simulink library "Lib_Piccolo"  (R2018b)
settings: Solver=VariableStepAuto  StartTime=0.0  StopTime=10.0  RelTol=1e-3
values from neighbouring files (symbols this model uses):
  AccelErrInt2Brakes = 0.15    [SimulationControlConfig16P.m]    (also in SimulationControlConfig16P_LEGACY.m; SimulationControlConfigTAILLESS.m = 0.2; SimulationControlConfigUTAIL.m = 0.2)
  AileronMax = 25    [SimulationControlConfig16P.m]    (also in SimulationControlConfig16P_LEGACY.m; SimulationControlConfigTAILLESS.m; SimulationControlConfigUTAIL.m)
  AileronPower = 0.00268    [SimulationControlConfig16P.m]    (also in SimulationControlConfig16P_LEGACY.m; SimulationControlConfigTAILLESS.m; SimulationControlConfigUTAIL.m)
  AileronSurfaceMax = 45    [SimulationControlConfig16P.m]    (also in SimulationControlConfig16P_LEGACY.m)
  AileronTrim = 0    [SimulationControlConfig16P.m]    (also in SimulationControlConfig16P_LEGACY.m; SimulationControlConfigTAILLESS.m; SimulationControlConfigUTAIL.m)
  Alt = 1000 + TerrainHeight    [SimulationStateConfig.m]
  AltCruise_m = testPlans(testIndx).terrainElevation * 0.3048 + 200    [SimulationControlConfig16P.m]    (also in SimulationControlConfigTAILLESS.m = 1083; SimulationControlConfigUTAIL.m = testPlans(testIndx).terrainElevation * 0.3048 + 152)
  AltitudeRate2PitchCmdIntegratorInit = 0.1    [SimulationControlPre.m]
  AltMax = 10000    [SimulationControlConfig16P.m]    (also in SimulationControlConfig16P_LEGACY.m; SimulationControlConfigTAILLESS.m; SimulationControlConfigUTAIL.m)
  AltMaxAccel = 1.25    [SimulationControlConfig16P.m]    (also in SimulationControlConfig16P_LEGACY.m = 0.9; SimulationControlConfigTAILLESS.m = 1.7; SimulationControlConfigUTAIL.m = 2)
  AltMin = 0    [SimulationControlConfig16P.m]    (also in SimulationControlConfig16P_LEGACY.m; SimulationControlConfigTAILLESS.m; SimulationControlConfigUTAIL.m)
  AltRateCmd2Pitch = 0.50    (= 0.5)    [SimulationControlConfig16P.m]    (also in SimulationControlConfig16P_LEGACY.m = 0.6; SimulationControlConfigTAILLESS.m = 0.2; SimulationControlConfigUTAIL.m = 0.3)
  AltRateError2Pitch = 0.40    (= 0.4)    [SimulationControlConfig16P.m]    (also in SimulationControlConfig16P_LEGACY.m; SimulationControlConfigTAILLESS.m = 0.55; SimulationControlConfigUTAIL.m = 0.55)
  AltRateErrorInt2Pitch = 0.50    (= 0.5)    [SimulationControlConfig16P.m]    (also in SimulationControlConfig16P_LEGACY.m = 0.45; SimulationControlConfigTAILLESS.m; SimulationControlConfigUTAIL.m = 0.75)
  AltRateLpfCutOff = 3    [SimulationControlConfig16P.m]    (also in SimulationControlConfig16P_LEGACY.m; SimulationControlConfigTAILLESS.m = 2; SimulationControlConfigUTAIL.m = 2)
  AutoNosegear2Rudder = 26    [SimulationControlConfig16P.m]    (also in SimulationControlConfig16P_LEGACY.m; SimulationControlConfigTAILLESS.m = 25.2; SimulationControlConfigUTAIL.m = 14)
  b = 5.54    [SimulationControlConfig16P.m]    (also in SimulationControlConfig16P_LEGACY.m; SimulationControlConfigTAILLESS.m = 2.37; SimulationControlConfigUTAIL.m = 2.37)
  Bank2AileronIntegratorInit = 0    [SimulationControlPre.m]
  BankMax_User = BankMax_User/180*pi    (= 0.523598775598)    [SimulationControlConfig16P.m]    (also in SimulationControlConfig16P_LEGACY.m; SimulationControlConfigTAILLESS.m = 0.610865238198; SimulationControlConfigUTAIL.m = 0.628318530718)
  baseLegFlaps = 20    [SimulationControlConfig16P.m]    (also in SimulationControlConfig16P_LEGACY.m = 0; SimulationControlConfigTAILLESS.m = 15; SimulationControlConfigUTAIL.m = 10)
  C = GeneticOpt.C    [SimulationCostFunction.m]
  c = Sw/b    (= 0.841696750903)    [SimulationControlConfig16P.m]    (also in SimulationControlConfig16P_LEGACY.m; SimulationControlConfigTAILLESS.m = 0.354008438819; SimulationControlConfigUTAIL.m = 0.354008438819)
  cell2WheelFactorMG = 5.98    [SimulationSensorConfig16P_LEGACY.m]
  cell2WheelFactorNG = 1    [SimulationSensorConfig16P_LEGACY.m]
  cellSatMaxMG = 15000    [SimulationSensorConfig16P.m]    (also in SimulationSensorConfig16P_LEGACY.m; SimulationSensorConfigTAILLESS7P.m; SimulationSensorConfigUTAIL7P.m)
  cellSatMaxNG = 1000    [SimulationSensorConfig16P.m]    (also in SimulationSensorConfig16P_LEGACY.m; SimulationSensorConfigTAILLESS7P.m; SimulationSensorConfigUTAIL7P.m)
  cellSatMinMG = -15000    [SimulationSensorConfig16P.m]    (also in SimulationSensorConfig16P_LEGACY.m; SimulationSensorConfigTAILLESS7P.m; SimulationSensorConfigUTAIL7P.m)
  cellSatMinNG = -1000    [SimulationSensorConfig16P.m]    (also in SimulationSensorConfig16P_LEGACY.m; SimulationSensorConfigTAILLESS7P.m; SimulationSensorConfigUTAIL7P.m)
  CL_Limit = CL_Max    (= 0.54)    [SimulationControlConfig16P.m]    (also in SimulationControlConfig16P_LEGACY.m; SimulationControlConfigTAILLESS.m; SimulationControlConfigUTAIL.m = 0.53)
  CL_Max = 0.54    [SimulationControlConfig16P.m]    (also in SimulationControlConfig16P_LEGACY.m; SimulationControlConfigTAILLESS.m; SimulationControlConfigUTAIL.m = 0.53)
  CL_Max_Nom = 0.465    [SimulationControlConfig16P.m]    (also in SimulationControlConfig16P_LEGACY.m; SimulationControlConfigTAILLESS.m = 0.39; SimulationControlConfigUTAIL.m)
  CL_Min = 0    [SimulationControlConfig16P.m]    (also in SimulationControlConfig16P_LEGACY.m; SimulationControlConfigTAILLESS.m; SimulationControlConfigUTAIL.m)
  ClimbMaxFraction = 0.35    [SimulationControlConfig16P.m]    (also in SimulationControlConfig16P_LEGACY.m = 0.24; SimulationControlConfigTAILLESS.m = 0.19; SimulationControlConfigUTAIL.m = 0.21)
  ClimboutMaxBank = 7.0    (= 7)    [SimulationControlConfig16P.m]    (also in SimulationControlConfig16P_LEGACY.m; SimulationControlConfigTAILLESS.m = 5; SimulationControlConfigUTAIL.m)
  ClimboutTimer = 7.0    (= 7)    [SimulationControlConfig16P.m]    (also in SimulationControlConfig16P_LEGACY.m; SimulationControlConfigTAILLESS.m; SimulationControlConfigUTAIL.m)
  dCl_per_dFlap = 0.005581818    [SimulationControlConfig16P.m]    (also in SimulationControlConfig16P_LEGACY.m = 0; SimulationControlConfigTAILLESS.m = 0; SimulationControlConfigUTAIL.m = 0)
  DecelerationCmd = 3.1    [SimulationControlConfig16P.m]    (also in SimulationControlConfig16P_LEGACY.m; SimulationControlConfigTAILLESS.m = 0.1; SimulationControlConfigUTAIL.m = 0.1)
  DeRotateLogicEndTimer = abs((NoseDownLimit_Deg-1)/DeRotateRamp_Dps)    [SimulationControlConfig16P.m]    (also in SimulationControlConfig16P_LEGACY.m; SimulationControlConfigTAILLESS.m; SimulationControlConfigUTAIL.m)
  DeRotateLogicHoldNoseUpTimer = 0.1    [SimulationControlConfig16P.m]    (also in SimulationControlConfig16P_LEGACY.m; SimulationControlConfigTAILLESS.m; SimulationControlConfigUTAIL.m)
  DeRotateLogicTimerTimeout = 2    [SimulationControlConfig16P.m]    (also in SimulationControlConfig16P_LEGACY.m; SimulationControlConfigTAILLESS.m; SimulationControlConfigUTAIL.m)
  DeRotateLowerCmdSaturation = 0    [SimulationControlConfig16P.m]    (also in SimulationControlConfig16P_LEGACY.m; SimulationControlConfigTAILLESS.m; SimulationControlConfigUTAIL.m)
  DeRotateRamp_Dps = 3    [SimulationControlConfig16P.m]    (also in SimulationControlConfig16P_LEGACY.m; SimulationControlConfigTAILLESS.m = 8; SimulationControlConfigUTAIL.m = 8)
  DeRotateUpperCmdSaturation = 7    [SimulationControlConfig16P.m]    (also in SimulationControlConfig16P_LEGACY.m; SimulationControlConfigTAILLESS.m; SimulationControlConfigUTAIL.m)
  DescentMaxFraction = 0.22    [SimulationControlConfig16P.m]    (also in SimulationControlConfig16P_LEGACY.m = 0.2; SimulationControlConfigTAILLESS.m = 0.17; SimulationControlConfigUTAIL.m = 0.17)
  DesktopSimTerrainOffset_m = 0.406    [SimulationAircraftConfig.m]
  downwindFlaps = 0    [SimulationControlConfig16P.m]    (also in SimulationControlConfig16P_LEGACY.m; SimulationControlConfigTAILLESS.m; SimulationControlConfigUTAIL.m)
  DP_init = 0.5*1.225*V_init^2    [SimulationControlConfig16P.m]    (also in SimulationControlConfig16P_LEGACY.m; SimulationControlConfigTAILLESS.m; SimulationControlConfigUTAIL.m)
  dscNoiseMG = 1    [SimulationSensorConfig16P_LEGACY.m]
  dscNoiseNG = 0.25    [SimulationSensorConfig16P_LEGACY.m]
  DSCnumBits = 24    [SimulationSensorConfig16P.m]    (also in SimulationSensorConfig16P_LEGACY.m; SimulationSensorConfigTAILLESS7P.m; SimulationSensorConfigUTAIL7P.m)
  DSCRangeMaxMG = 15000    [SimulationSensorConfig16P.m]    (also in SimulationSensorConfig16P_LEGACY.m; SimulationSensorConfigTAILLESS7P.m; SimulationSensorConfigUTAIL7P.m)
  DSCRangeMaxNG = 1000    [SimulationSensorConfig16P.m]    (also in SimulationSensorConfig16P_LEGACY.m; SimulationSensorConfigTAILLESS7P.m; SimulationSensorConfigUTAIL7P.m)
  DSCRangeMinMG = -15000    [SimulationSensorConfig16P.m]    (also in SimulationSensorConfig16P_LEGACY.m; SimulationSensorConfigTAILLESS7P.m; SimulationSensorConfigUTAIL7P.m)
  DSCRangeMinNG = -1000    [SimulationSensorConfig16P.m]    (also in SimulationSensorConfig16P_LEGACY.m; SimulationSensorConfigTAILLESS7P.m; SimulationSensorConfigUTAIL7P.m)
  dt = DLLSim.dt    [SimulationTimeStep.m]    (also in SimulationTrim.m = 0.02)
  EarlyTouchdownThreshold = 3.0    (= 3)    [SimulationControlConfig16P.m]    (also in SimulationControlConfig16P_LEGACY.m; SimulationControlConfigTAILLESS.m = 2.2; SimulationControlConfigUTAIL.m = 2.5)
  ElevatorDeflectionRate = 15    [SimulationControlConfig16P.m]    (also in SimulationControlConfig16P_LEGACY.m = 12; SimulationControlConfigTAILLESS.m = 10; SimulationControlConfigUTAIL.m = 12)
  ElevatorMax = 25    [SimulationControlConfig16P.m]    (also in SimulationControlConfig16P_LEGACY.m; SimulationControlConfigTAILLESS.m; SimulationControlConfigUTAIL.m)
  ElevatorPower = -0.002209    [SimulationControlConfig16P.m]    (also in SimulationControlConfig16P_LEGACY.m; SimulationControlConfigTAILLESS.m = -0.002956; SimulationControlConfigUTAIL.m = -0.00205983)
  ElevatorTrim = -3.5    [SimulationControlConfig16P.m]    (also in SimulationControlConfig16P_LEGACY.m; SimulationControlConfigTAILLESS.m = -6; SimulationControlConfigUTAIL.m = -8)
  elevonBias = 0    [SimulationControlConfig16P.m]    (also in SimulationControlConfig16P_LEGACY.m; SimulationControlConfigTAILLESS.m; SimulationControlConfigUTAIL.m)
  Enable_TAS_Protection = 0    [SimulationControlConfig16P.m]    (also in SimulationControlConfig16P_LEGACY.m; SimulationControlConfigTAILLESS.m; SimulationControlConfigUTAIL.m)
  EnableCrossTrackAbort = 1    [SimulationControlConfig16P.m]    (also in SimulationControlConfigTAILLESS.m; SimulationControlConfigUTAIL.m)
  EnergyBandwidth = 0.02    [SimulationControlConfig16P.m]    (also in SimulationControlConfig16P_LEGACY.m; SimulationControlConfigTAILLESS.m = 0.06; SimulationControlConfigUTAIL.m = 0.06)
  EngineLhFuelCut = 0    [SimulationAircraftConfig.m]
  EngineRhFuelCut = 0    [SimulationAircraftConfig.m]
  FastThrottleRate = 0.075    [SimulationControlConfig16P.m]    (also in SimulationControlConfig16P_LEGACY.m = 0.05; SimulationControlConfigTAILLESS.m = 0.1; SimulationControlConfigUTAIL.m = 0.1)
  FilterWarmUpTime = 2    [SimulationSensorConfig16P.m]    (also in SimulationSensorConfig16P_LEGACY.m; SimulationSensorConfigTAILLESS7P.m; SimulationSensorConfigUTAIL7P.m)
  finalApproachFlaps = 20    [SimulationControlConfig16P.m]    (also in SimulationControlConfig16P_LEGACY.m = 0; SimulationControlConfigTAILLESS.m = 22; SimulationControlConfigUTAIL.m = 10)
  FinalDescentSlope_Deg = testPlans(testIndx).descentSlope    [SimulationControlConfig16P.m]    (also in SimulationControlConfig16P_LEGACY.m; SimulationControlConfigTAILLESS.m; SimulationControlConfigUTAIL.m)
  flapMax = 0    [SimulationControlConfig16P.m]    (also in SimulationControlConfig16P_LEGACY.m; SimulationControlConfigTAILLESS.m; SimulationControlConfigUTAIL.m)
  flapRate = 7.5    [SimulationControlConfig16P.m]    (also in SimulationControlConfig16P_LEGACY.m; SimulationControlConfigTAILLESS.m = 6.6; SimulationControlConfigUTAIL.m)
  FlareHeight = 5    [SimulationControlConfig16P.m]    (also in SimulationControlConfig16P_LEGACY.m = 4.8; SimulationControlConfigTAILLESS.m = 2.5; SimulationControlConfigUTAIL.m = 2)
  FlareVerticalRate_mps = -0.4    [SimulationControlConfig16P.m]    (also in SimulationControlConfig16P_LEGACY.m = -0.5; SimulationControlConfigTAILLESS.m = -0.15; SimulationControlConfigUTAIL.m = -0.15)
  Fp_Aileron = 0.55*2*pi*RollRateLpfCutoff*dt    [SimulationControlConfig16P.m]    (also in SimulationControlConfig16P_LEGACY.m; SimulationControlConfigTAILLESS.m; SimulationControlConfigUTAIL.m)
  Fp_Alt = 0.55*AltBandwidth    (= 0.099)    [SimulationControlConfig16P.m]    (also in SimulationControlConfig16P_LEGACY.m; SimulationControlConfigTAILLESS.m = 0.587477826221; SimulationControlConfigUTAIL.m = 0.69115038379)
  Fp_AltRate = 0.55*2*pi*AltRateLpfCutOff*dt    [SimulationControlConfig16P.m]    (also in SimulationControlConfig16P_LEGACY.m; SimulationControlConfigTAILLESS.m; SimulationControlConfigUTAIL.m)
  Fp_Elevator = 0.55*2*pi*PitchRateLpfCutoff*dt    [SimulationControlConfig16P.m]    (also in SimulationControlConfig16P_LEGACY.m; SimulationControlConfigTAILLESS.m; SimulationControlConfigUTAIL.m)
  Fp_Energy = 0.55*2*pi*EnergyBandwidth    (= 0.069115038379)    [SimulationControlConfig16P.m]    (also in SimulationControlConfig16P_LEGACY.m; SimulationControlConfigTAILLESS.m = 0.207345115137; SimulationControlConfigUTAIL.m = 0.207345115137)
  Fp_Energy2 = 0.55*2*pi*EnergyBandwidth*dt    [SimulationControlConfig16P.m]    (also in SimulationControlConfig16P_LEGACY.m; SimulationControlConfigTAILLESS.m; SimulationControlConfigUTAIL.m)
  Fp_Pitch = 0.55*2*pi*PitchBandwidth    (= 2.76460153516)    [SimulationControlConfig16P.m]    (also in SimulationControlConfig16P_LEGACY.m = 3.11017672705; SimulationControlConfigTAILLESS.m = 3.80132711084; SimulationControlConfigUTAIL.m = 2.41902634326)
  Fp_Pitch_2 = 0.55*2*pi*PitchBandwidth*dt    [SimulationControlConfig16P.m]    (also in SimulationControlConfig16P_LEGACY.m; SimulationControlConfigTAILLESS.m; SimulationControlConfigUTAIL.m)
  Fp_Roll = RollBandwidth^2    (= 1)    [SimulationControlConfig16P.m]    (also in SimulationControlConfig16P_LEGACY.m = 1.44; SimulationControlConfigTAILLESS.m; SimulationControlConfigUTAIL.m)
  Fp_Rudder = 0.55*2*pi*YawRateLpfCutoff*dt    [SimulationControlConfig16P.m]    (also in SimulationControlConfig16P_LEGACY.m; SimulationControlConfigTAILLESS.m; SimulationControlConfigUTAIL.m)
  Fp_TAS = 0.55*2*pi*TASBandwidth    (= 0.103672557568)    [SimulationControlConfig16P.m]    (also in SimulationControlConfig16P_LEGACY.m; SimulationControlConfigTAILLESS.m = 0.172787595947; SimulationControlConfigUTAIL.m = 0.172787595947)
  Fp_TAS_Filter = 2*pi*TasLpfCutoff*dt    [SimulationControlConfig16P.m]    (also in SimulationControlConfig16P_LEGACY.m; SimulationControlConfigTAILLESS.m; SimulationControlConfigUTAIL.m)
  Fp_Turn = 0.55*2*pi*TurnErrLPFcutoff    (= 0.0345575191895)    [SimulationControlConfig16P.m]    (also in SimulationControlConfig16P_LEGACY.m; SimulationControlConfigTAILLESS.m = 0.172787595947; SimulationControlConfigUTAIL.m = 0.172787595947)
  Fp_TurnDerr = 0.55*2*pi*TurnDerivativeLPFcutoff    (= 0.0345575191895)    [SimulationControlConfig16P.m]    (also in SimulationControlConfig16P_LEGACY.m; SimulationControlConfigTAILLESS.m = 0.172787595947; SimulationControlConfigUTAIL.m = 0.172787595947)
  FTV = 3    [SimulationAircraftConfig.m]
  ftvStaticPositionError = 1/1.18    (= 0.847457627119)    [SimulationSensorConfig16P.m]    (also in SimulationSensorConfig16P_LEGACY.m; SimulationSensorConfigTAILLESS7P.m = 1; SimulationSensorConfigUTAIL7P.m = 1)
  g = 9.81    [SimulationStateConfig.m]
  GustSpd_Kts = testPlans(testIndx).gustSpd    [SimulationStateConfig.m]
  GustTriggerVal = testPlans(testIndx).gustTriggerVal    [SimulationStateConfig.m]
  HeadingErr2TurnRate = 0.5    [SimulationControlConfig16P.m]    (also in SimulationControlConfig16P_LEGACY.m; SimulationControlConfigTAILLESS.m; SimulationControlConfigUTAIL.m)
  HeadingErrDer2TurnRate = 0.3    [SimulationControlConfig16P.m]    (also in SimulationControlConfig16P_LEGACY.m; SimulationControlConfigTAILLESS.m; SimulationControlConfigUTAIL.m)
  IASbounce = IASstall*0.8    [SimulationControlPre.m]
  IAScruiseCMD = sqrt(2*m*9.81/(1.225*Sw*CL_cruise))    [SimulationControlConfig16P.m]    (also in SimulationControlConfig16P_LEGACY.m; SimulationControlConfigTAILLESS.m; SimulationControlConfigUTAIL.m)
  IASfinalCMD = 1.12 * IASmin    [SimulationControlConfig16P.m]    (also in SimulationControlConfig16P_LEGACY.m = 1.10 * IASmin; SimulationControlConfigTAILLESS.m = 1.10 * IASmin; SimulationControlConfigUTAIL.m = 1.15 * IASmin)
  IASflareCMD = IASstall    [SimulationControlConfig16P.m]    (also in SimulationControlConfig16P_LEGACY.m; SimulationControlConfigTAILLESS.m; SimulationControlConfigUTAIL.m)
  IASmax = 64    [SimulationControlConfig16P.m]    (also in SimulationControlConfig16P_LEGACY.m = 46; SimulationControlConfigTAILLESS.m = 38.58; SimulationControlConfigUTAIL.m = 35)
  IASmin = sqrt(2*m*9.81/(1.225*Sw*0.9*CL_Max_Nom))    [SimulationControlConfig16P.m]    (also in SimulationControlConfig16P_LEGACY.m; SimulationControlConfigTAILLESS.m; SimulationControlConfigUTAIL.m)
  IASshortCMD = IASstall    [SimulationControlConfig16P.m]    (also in SimulationControlConfig16P_LEGACY.m; SimulationControlConfigTAILLESS.m; SimulationControlConfigUTAIL.m)
  IASstall = sqrt(2*m*9.81/(1.225*Sw*CL_Max))    [SimulationControlConfig16P.m]    (also in SimulationControlConfig16P_LEGACY.m; SimulationControlConfigTAILLESS.m; SimulationControlConfigUTAIL.m)
  inFlight = 1    [SimulationControlConfig16P.m]    (also in SimulationControlConfigTAILLESS.m; SimulationControlConfigUTAIL.m)
  JetCatOffset = 5    [SimulationControlConfig16P.m]    (also in SimulationControlConfig16P_LEGACY.m)
  LaunchRollingElevator = -1.5    [SimulationControlConfig16P.m]    (also in SimulationControlConfig16P_LEGACY.m; SimulationControlConfigTAILLESS.m = 1; SimulationControlConfigUTAIL.m = 1)
  ldg_NosegearMax = 10    [SimulationControlConfig16P.m]    (also in SimulationControlConfig16P_LEGACY.m; SimulationControlConfigTAILLESS.m; SimulationControlConfigUTAIL.m)
  ldg_TrackVyErrInt2Nosegear = 0.1250    (= 0.125)    [SimulationControlConfig16P.m]    (also in SimulationControlConfig16P_LEGACY.m; SimulationControlConfigTAILLESS.m = 0.00714285714286; SimulationControlConfigUTAIL.m = 0.00714285714286)
  ldg_TrackVyErrPro2Nosegear = 0.35    [SimulationControlConfig16P.m]    (also in SimulationControlConfig16P_LEGACY.m; SimulationControlConfigTAILLESS.m = 0.0546666666667; SimulationControlConfigUTAIL.m = 0.0546666666667)
  ldg_TrackY2Vy = 0.07    [SimulationControlConfig16P.m]    (also in SimulationControlConfig16P_LEGACY.m; SimulationControlConfigTAILLESS.m = 0.17; SimulationControlConfigUTAIL.m = 0.17)
  ldg_Vy2NosegearScalingPower = 1.075    [SimulationControlConfig16P.m]    (also in SimulationControlConfig16P_LEGACY.m; SimulationControlConfigTAILLESS.m = 0.6; SimulationControlConfigUTAIL.m = 0.5)
  ldg_Y2VyScalingPower = 0.175    [SimulationControlConfig16P.m]    (also in SimulationControlConfig16P_LEGACY.m; SimulationControlConfigTAILLESS.m = 0; SimulationControlConfigUTAIL.m = 0)
  ldg_YawRate2Nosegear = 0.175    [SimulationControlConfig16P.m]    (also in SimulationControlConfig16P_LEGACY.m; SimulationControlConfigTAILLESS.m = 0.065; SimulationControlConfigUTAIL.m = 0.065)
  LiftSlope = 0.064285    [SimulationControlConfig16P.m]    (also in SimulationControlConfig16P_LEGACY.m; SimulationControlConfigTAILLESS.m = 0.058631; SimulationControlConfigUTAIL.m)
  LPFaileronInit = 0    [SimulationControlPre.m]
  LPFclestInit = 0    [SimulationControlPre.m]
  LPFenergyFFInit = 0    [SimulationControlPre.m]
  LPFtasInit = V_init + 2    [SimulationControlPre.m]
  LPFthrottleInit = ThrottleTrim    [SimulationControlPre.m]
  LPFturnErrInit = 0    [SimulationControlPre.m]
  ... (+115 more)
undefined symbols (not defined in the file or in its folder): abortFlag, alphaHPF, apmDelay, BRWNOUT, CRAWOR, CRAWUR, DiscIntNeverNeededParam, DLLSim, DLLSimStep, ECOMOR, ECOMUR, Fp_Tas, GustTrigger_HeightAgl_m, IPSTAT, LCINTEG, Ldg_Persist_Time, LOWER_FLAGS, MSG_ENABLE, NoiseStd, OLDVAL, OVERRIDE_ENABLE, OVERRIDE_VALUE, REBOOT, reversionEnable, revIASMax, revIASMin, revPitchMax, revPitchMin, revPitchRateMax, revRollMax, revRollRateMax, SAMPLE, SCALON, SensorModel, sigbuilder_block, Sim_Vx, Sim_Vy, Sim_Vz, Sim_Xpos, Sim_Ypos, Sim_Zpos, SYSOR, SYSUR, TARE, TEMPOR, TEMPUR, testIndx, testPlan, testPlans, Trim_piccoloInCmd, Trim_REFSI_FD_IN_nmodeCgShifterCmd_Ft, Trim_REFSI_FD_IN_nmodeFlapLhIBCmd_Deg, Trim_REFSI_FD_IN_nmodeFlapLhOBCmd_Deg, Trim_REFSI_FD_IN_nmodeFlapRhIBCmd_Deg, Trim_REFSI_FD_IN_nmodeFlapRhOBCmd_Deg, Trim_REFSI_FD_IN_nmodeSlatLhCmd_Deg, Trim_REFSI_FD_IN_nmodeSlatRhCmd_Deg, Trim_REFSI_FD_IN_nmodeSplrLhInbdCmd_Deg, Trim_REFSI_FD_IN_nmodeSplrLhOutbdCmd_Deg ... (+5)
libraries: simulink x866, aerolibconvert2 x60, $bdroot x52, aerolibatmos2 x5, dspswit3 x5, simulink_extras x4, dsparch4 x2, Lib_Piccolo_Alt x2, eeGeneralControl x1, dspindex x1
(part 40 of 44)

== system Lib_Piccolo/Ground Detection Systems/WoW Wrapper/Variant Subsystem/Load Cell WoW Model 20/WOW Module/Bias Filters ==
  WOW_NG_RAW_N : Inport
  WOW_MGL_RAW_N : Inport  Port=2
  WOW_MGR_RAW_N : Inport  Port=3
  Bus Creator : BusCreator  Inputs=3
  Ground : Ground
  LPF MGL : Subsystem  mask{Cutoff=SensorModel.WOW.Cell.fc, Init=0}
      mask prompts: Cutoff "Cutoff Frequency [Hz]"; Init "Initial Condition"
  LPF MGR : Subsystem  mask{Cutoff=SensorModel.WOW.Cell.fc, Init=0}
      mask prompts: Cutoff "Cutoff Frequency [Hz]"; Init "Initial Condition"
  LPF NG : Subsystem  mask{Cutoff=SensorModel.WOW.Cell.fc, Init=0}
      mask prompts: Cutoff "Cutoff Frequency [Hz]"; Init "Initial Condition"
  WOW_Bias_Filt_N : Outport  VectorParamsAs1DForOutWhenUnconnected=on
  wires:
  WOW_NG_RAW_N/1 -> LPF NG/1("Input ")
  Bus Creator/1 -> WOW_Bias_Filt_N/1
  LPF NG/1("Output ") -> Bus Creator/1  "Bias_NG_N"
  Ground/1 -> LPF MGL/2(Reset), LPF MGR/2(Reset), LPF NG/2(Reset)
  WOW_MGL_RAW_N/1 -> LPF MGL/1("Input ")
  LPF MGL/1("Output ") -> Bus Creator/2  "Bias_MGL_N"
  LPF MGR/1("Output ") -> Bus Creator/3  "Bias_MGR_N"
  WOW_MGR_RAW_N/1 -> LPF MGR/1("Input ")

== system Lib_Piccolo/Ground Detection Systems/WoW Wrapper/Variant Subsystem/Load Cell WoW Model 20/WOW Module/Command Processing ==
  User Cmd Bus In : Inport
  Bus Selector : BusSelector  OutputSignals=MSG_ENABLE,TARE,OVERRIDE_ENABLE,OVERRIDE_VALUE
  Edge Detector : dspswit3/Edge Detector  InputProcessing=Columns as channels (frame based)
      settings: SourceProductName=DSP System Toolbox  SourceProductBaseCode=DS
  TARE_TRIGGER : Outport
  MSG_ENABLE : Outport  Port=2
  OVERRIDE_ENABLE : Outport  Port=3  OutDataTypeStr=boolean  VectorParamsAs1DForOutWhenUnconnected=on
  OVERRIDE_VALUE : Outport  Port=4  OutDataTypeStr=boolean  VectorParamsAs1DForOutWhenUnconnected=on
  User Cmd Bus Out : Outport  Port=5
  wires:
  Bus Selector/1 -> MSG_ENABLE/1  "<MSG_ENABLE>"
  User Cmd Bus In/1 -> Bus Selector/1, User Cmd Bus Out/1
  Bus Selector/2 -> Edge Detector/1  "<TARE>"
  Edge Detector/1 -> TARE_TRIGGER/1
  Bus Selector/3 -> OVERRIDE_ENABLE/1  "<OVERRIDE_ENABLE>"
  Bus Selector/4 -> OVERRIDE_VALUE/1  "<OVERRIDE_VALUE>"

== system Lib_Piccolo/Ground Detection Systems/WoW Wrapper/Variant Subsystem/Load Cell WoW Model 20/WOW Module/Flag Latch ==
  note: Latch failure/disable state if AP mode is <= climbout, or >= final
  INIT : Inport
  OUTPUT_DISABLE : Inport  Port=2
  PIC_AP_MODE : Inport  Port=3
  Latch : Subsystem
  Latch Activation on Mode : Subsystem
  OR5 : Logic  Operator=OR  IconShape=distinctive  AllPortsSameDT=off  OutDataTypeStr=boolean
  OUTPUT_DISABLE_LATCHED : Outport
  wires:
  INIT/1 -> OR5/1
  Latch/1(Q_Latched) -> OUTPUT_DISABLE_LATCHED/1
  OUTPUT_DISABLE/1 -> OR5/2
  OR5/1 -> Latch/1(D)
  PIC_AP_MODE/1 -> Latch Activation on Mode/1(Piccolo Mode)
  Latch Activation on Mode/1(Mode Latch) -> Latch/2(Enable/!Rst)

== system Lib_Piccolo/Ground Detection Systems/WoW Wrapper/Variant Subsystem/Load Cell WoW Model 20/WOW Module/LPF MGL ==
  "Input " : Inport
  Reset : Inport  Port=2
  Add1 : Sum  Inputs=++|
  Compare To Constant2 : simulink/Logic and Bit Operations/Compare To Constant  relop=>  const=0  OutDataTypeStr=uint8
  Constant11 : Constant  Value=Cutoff
  Resettable Delay : Delay  DelayLength=1  InitialConditionSource=Input port  ExternalReset=Level hold
      settings: InputPortMap=u0,r5,p4
  Switch1 : Switch  Criteria=u2 > Threshold
  a1 : Gain  Gain=SensorModel.WOW.Cell.a1
  b0 : Gain  Gain=SensorModel.WOW.Cell.b0
  "Output " : Outport
  wires:
  Resettable Delay/1 -> a1/1
  b0/1 -> Add1/2
  Add1/1 -> Resettable Delay/1, Switch1/1
  a1/1 -> Add1/1
  "Input "/1 -> b0/1, Switch1/3, Resettable Delay/3
  Switch1/1 -> "Output "/1
  Compare To Constant2/1 -> Switch1/2
  Constant11/1 -> Compare To Constant2/1
  Reset/1 -> Resettable Delay/2

== system Lib_Piccolo/Ground Detection Systems/WoW Wrapper/Variant Subsystem/Load Cell WoW Model 20/WOW Module/LPF MGR ==
  "Input " : Inport
  Reset : Inport  Port=2
  Add1 : Sum  Inputs=++|
  Compare To Constant2 : simulink/Logic and Bit Operations/Compare To Constant  relop=>  const=0  OutDataTypeStr=uint8
  Constant11 : Constant  Value=Cutoff
  Resettable Delay : Delay  DelayLength=1  InitialConditionSource=Input port  ExternalReset=Level hold
      settings: InputPortMap=u0,r5,p4
  Switch1 : Switch  Criteria=u2 > Threshold
  a1 : Gain  Gain=SensorModel.WOW.Cell.a1
  b0 : Gain  Gain=SensorModel.WOW.Cell.b0
  "Output " : Outport
  wires:
  Resettable Delay/1 -> a1/1
  b0/1 -> Add1/2
  Add1/1 -> Resettable Delay/1, Switch1/1
  a1/1 -> Add1/1
  "Input "/1 -> b0/1, Switch1/3, Resettable Delay/3
  Switch1/1 -> "Output "/1
  Compare To Constant2/1 -> Switch1/2
  Constant11/1 -> Compare To Constant2/1
  Reset/1 -> Resettable Delay/2

== system Lib_Piccolo/Ground Detection Systems/WoW Wrapper/Variant Subsystem/Load Cell WoW Model 20/WOW Module/LPF NG ==
  "Input " : Inport
  Reset : Inport  Port=2
  Add1 : Sum  Inputs=++|
  Compare To Constant2 : simulink/Logic and Bit Operations/Compare To Constant  relop=>  const=0  OutDataTypeStr=uint8
  Constant11 : Constant  Value=Cutoff
  Resettable Delay : Delay  DelayLength=1  InitialConditionSource=Input port  ExternalReset=Level hold
      settings: InputPortMap=u0,r5,p4
  Switch1 : Switch  Criteria=u2 > Threshold
  a1 : Gain  Gain=SensorModel.WOW.Cell.a1
  b0 : Gain  Gain=SensorModel.WOW.Cell.b0
  "Output " : Outport
  wires:
  Reset/1 -> Resettable Delay/2
  Constant11/1 -> Compare To Constant2/1
  Compare To Constant2/1 -> Switch1/2
  Switch1/1 -> "Output "/1
  "Input "/1 -> b0/1, Switch1/3, Resettable Delay/3
  a1/1 -> Add1/1
  Add1/1 -> Switch1/1, Resettable Delay/1
  b0/1 -> Add1/2
  Resettable Delay/1 -> a1/1

== system Lib_Piccolo/Ground Detection Systems/WoW Wrapper/Variant Subsystem/Load Cell WoW Model 20/WOW Module/Landing Configuration ==
  WOW_Filt : Inport
  DSC_Fail : Inport  Port=2
  AND1 : Logic  IconShape=distinctive  AllPortsSameDT=off  OutDataTypeStr=boolean
  Bus Selector : BusSelector  OutputSignals=WOW_Filt_NG_N,WOW_Filt_MGL_N,WOW_Filt_MGR_N
  Bus Selector1 : BusSelector  OutputSignals=MGR_DSC_FAIL,MGL_DSC_FAIL
  Enable : Constant  Value=SensorModel.WOW.Cell.useDualLogic
  Gain1 : Gain
  Gain2 : Gain
  Hysteresis L : Relay  OnSwitchValue=SensorModel.WOW.Cell.loadThresholdUpper_N  OffSwitchValue=SensorModel.WOW.Cell.loadThresholdLower_N
  Hysteresis R : Relay  OnSwitchValue=SensorModel.WOW.Cell.loadThresholdUpper_N  OffSwitchValue=SensorModel.WOW.Cell.loadThresholdLower_N
  Input Selection (Failure Handling) : Subsystem
  Latching Logic : Subsystem
  Logic Selection : Subsystem
  Persistance Timer : Subsystem  mask{period=SensorModel.WOW.Cell.persistanceTime_s}
      mask prompts: period "Period [s]"
  Terminator : Terminator
  Terminator1 : Terminator
  Terminator2 : Terminator
  Timeout Logic : Subsystem
  Unit Delay : UnitDelay  SampleTime=-1
  ContactBool : Outport
  Landing_Fail_L : Outport  Port=2
  Landing_Fail_R : Outport  Port=3
  wires:
  Enable/1 -> AND1/1
  AND1/1 -> Logic Selection/2(Logic Mode (Or/!And)), Timeout Logic/2(Logic Mode (Or/!And))  "Logic Mode (Or/!And)"
  [Contact] -> AND1/2
  Bus Selector/1 -> Terminator/1  "<WOW_Filt_NG_N>"
  WOW_Filt/1 -> Bus Selector/1
  Gain2/1 -> Terminator2/1  "ContactR"
  Gain1/1 -> Terminator1/1  "ContactL"
  Hysteresis R/1 -> Gain2/1, Logic Selection/3(ContactR), Timeout Logic/3(ContactR)
  Hysteresis L/1 -> Timeout Logic/1(ContactL), Logic Selection/1(ContactL), Gain1/1
  Unit Delay/1 -> [Contact]
  Latching Logic/1(ContactOut) -> ContactBool/1, Unit Delay/1  "ContactBool"
  DSC_Fail/1 -> Bus Selector1/1
  Input Selection (Failure Handling)/2(InputR) -> Hysteresis R/1  "InputR"
  Input Selection (Failure Handling)/1(InputL) -> Hysteresis L/1  "InputL"
  Persistance Timer/1(Expired) -> Latching Logic/1(ContactIn)
  Bus Selector/2 -> Input Selection (Failure Handling)/1(WOW_Filt_MGL_N)  "<WOW_Filt_MGL_N>"
  Bus Selector/3 -> Input Selection (Failure Handling)/2(WOW_Filt_MGR_N)  "<WOW_Filt_MGR_N>"
  Bus Selector1/1 -> Input Selection (Failure Handling)/3(MGR_DSC_FAIL)  "<MGR_DSC_FAIL>"
  Bus Selector1/2 -> Input Selection (Failure Handling)/4(MGL_DSC_FAIL)  "<MGL_DSC_FAIL>"
  Logic Selection/1(ContactOut) -> Persistance Timer/1(Enable/!Rst)
  Input Selection (Failure Handling)/4(FailR) -> Landing_Fail_R/1
  Input Selection (Failure Handling)/3(FailL) -> Landing_Fail_L/1

== system Lib_Piccolo/Ground Detection Systems/WoW Wrapper/Variant Subsystem/Load Cell WoW Model 20/WOW Module/Override Logic ==
  Logic Contact : Inport
  Override Enable : Inport  Port=2
  Override Value : Inport  Port=3
  Constant : Constant  Value=100  OutDataTypeStr=uint8
  Constant1 : Constant  Value=0  OutDataTypeStr=uint8
  Switch : Switch  Criteria=u2 > Threshold  Threshold=0.5
  Switch1 : Switch  Criteria=u2 > Threshold  Threshold=0.5
  CONTACT : Outport  VectorParamsAs1DForOutWhenUnconnected=on
  WOW_PCNT : Outport  Port=2  OutDataTypeStr=uint8  VectorParamsAs1DForOutWhenUnconnected=on
  wires:
  Override Enable/1 -> Switch/2
  Switch/1 -> Switch1/2, CONTACT/1
  Override Value/1 -> Switch/1
  Logic Contact/1 -> Switch/3
  Switch1/1 -> WOW_PCNT/1
  Constant/1 -> Switch1/1
  Constant1/1 -> Switch1/3

== system Lib_Piccolo/Ground Detection Systems/WoW Wrapper/Variant Subsystem/Load Cell WoW Model 20/WOW Module/Subsystem ==
  WOW_Bus : Inport
  MGR FLAG Word : Inport  Port=2
  MGR STAT Word : Inport  Port=3
  MGL FLAG Word : Inport  Port=4
  MGL STAT Word : Inport  Port=5
  NG FLAG Word : Inport  Port=6
  NG STAT Word : Inport  Port=7
  MGR_STALE_LOAD : Inport  Port=8  OutDataTypeStr=boolean
  MGR_STALE_FLAGS : Inport  Port=9  OutDataTypeStr=boolean
  MGL_STALE_LOAD : Inport  Port=10  OutDataTypeStr=boolean
  MGL_STALE_FLAGS : Inport  Port=11  OutDataTypeStr=boolean
  NG_STALE_LOAD : Inport  Port=12  OutDataTypeStr=boolean
  NG_STALE_FLAGS : Inport  Port=13  OutDataTypeStr=boolean
  NRC Active : Inport  Port=14
  PIC_AP_MODE : Inport  Port=15  OutDataTypeStr=uint8
  INIT : Inport  Port=16
  " Output Formatting" : Subsystem
  AND : Logic  Inputs=3  IconShape=distinctive  AllPortsSameDT=off  OutDataTypeStr=boolean
  AND1 : Logic  IconShape=distinctive  AllPortsSameDT=off
  AND2 : Logic  Inputs=3  IconShape=distinctive  AllPortsSameDT=off  OutDataTypeStr=boolean
  AND3 : Logic  Inputs=3  IconShape=distinctive  AllPortsSameDT=off  OutDataTypeStr=boolean
  Bus Assignment : BusAssignment  AssignedSignals=ACTIVE
  Bus Assignment1 : BusAssignment  AssignedSignals=ACTIVE
  Bus Assignment2 : BusAssignment  AssignedSignals=ACTIVE
  Bus Selector : BusSelector  OutputSignals=WOW_MGR_Filt_N,WOW_MGL_Filt_N,WOW_NG_Filt_N
  Comms Timeout Logic : Subsystem
  Health Check : Subsystem
  NOT : Logic  Operator=NOT  IconShape=distinctive  AllPortsSameDT=off  OutDataTypeStr=boolean
  MGR_DSC_FAIL : Outport  OutDataTypeStr=boolean
  MGL_DSC_FAIL : Outport  Port=2  OutDataTypeStr=boolean
  NG_DSC_FAIL : Outport  Port=3  OutDataTypeStr=boolean
  OUTPUT_DISABLE : Outport  Port=4
  NG_Out : Outport  Port=5
  MGL_Out : Outport  Port=6
  MGR_Out : Outport  Port=7
  wires:
  NOT/1 -> AND/2, AND2/2, AND3/2  "NRC_NOT_ACTIVE"
  Health Check/5(MGL_FLAGS) -> " Output Formatting"/5(MGL_FLAG)
  Health Check/2(MGL_FAIL) -> MGL_DSC_FAIL/1, AND1/2, AND2/1  "MGL_DSC_FAIL"
  Bus Selector/2 -> " Output Formatting"/14(MGL_WOW_Filt_N)  "<WOW_MGL_Filt_N>"
  Health Check/1(MGR_FAIL) -> MGR_DSC_FAIL/1, AND1/1, AND/1  "MGR_DSC_FAIL"
  Health Check/8(MGL_HEALTH) -> Bus Assignment1/1
  Health Check/4(MGR_FLAGS) -> " Output Formatting"/4(MGR_FLAG)
  Health Check/3(NG_FAIL) -> AND3/1, NG_DSC_FAIL/1  "NG_DSC_FAIL"
  Health Check/6(NG_FLAGS) -> " Output Formatting"/6(NG_FLAG)
  Bus Selector/3 -> " Output Formatting"/15(NG_WOW_Filt_N)  "<WOW_NG_Filt_N>"
  MGL FLAG Word/1 -> Health Check/4(MGL FLAG Word)
  NG STAT Word/1 -> Health Check/7(NG STAT Word)
  Health Check/9(NG_HEALTH) -> Bus Assignment2/1
  AND2/1 -> " Output Formatting"/2(MGL_RESET_REQUEST)  "RESET_REQUEST"
  Bus Selector/1 -> " Output Formatting"/13(MGR_WOW_Filt_N)  "<WOW_MGR_Filt_N>"
  AND/1 -> " Output Formatting"/1(MGR_RESET_REQUEST)  "RESET_REQUEST"
  NG FLAG Word/1 -> Health Check/6(NG FLAG Word)
  Health Check/7(MGR_HEALTH) -> Bus Assignment/1
  AND3/1 -> " Output Formatting"/3(NG_RESET_REQUEST)  "RESET_REQUEST"
  MGR FLAG Word/1 -> Health Check/2(MGR FLAG Word)
  WOW_Bus/1 -> Bus Selector/1, Health Check/14(WOW_N)
  MGR STAT Word/1 -> Health Check/3(MGR STAT Word)
  MGL STAT Word/1 -> Health Check/5(MGL STAT Word)
  NRC Active/1 -> NOT/1
  " Output Formatting"/2(MGL_Out) -> MGL_Out/1
  " Output Formatting"/3(MGR_Out) -> MGR_Out/1
  " Output Formatting"/1(NG_Out) -> NG_Out/1
  AND1/1 -> OUTPUT_DISABLE/1
  Health Check/10(MGR_STAT) -> " Output Formatting"/10(MGR_STAT)
  Health Check/11(MGL_STAT) -> " Output Formatting"/11(MGL_STAT)
  Health Check/12(NG_STAT) -> " Output Formatting"/12(NG_STAT)
  PIC_AP_MODE/1 -> Health Check/1(PIC_AP_MODE)
  MGR_STALE_LOAD/1 -> Comms Timeout Logic/1(MGR_STALE_LOAD)
  MGL_STALE_LOAD/1 -> Comms Timeout Logic/2(MGL_STALE_LOAD)
  NG_STALE_LOAD/1 -> Comms Timeout Logic/3(NG_STALE_LOAD)
  MGR_STALE_FLAGS/1 -> Comms Timeout Logic/4(MGR_STALE_FLAG)
  MGL_STALE_FLAGS/1 -> Comms Timeout Logic/5(MGL_STALE_FLAG)
  NG_STALE_FLAGS/1 -> Comms Timeout Logic/6(NG_STALE_FLAG)
  INIT/1 -> Comms Timeout Logic/7(INIT)
  Comms Timeout Logic/1(MGR_LOAD_TIMEOUT) -> Health Check/8(MGR_LOAD_TIMEOUT)
  Comms Timeout Logic/2(MGL_LOAD_TIMEOUT) -> Health Check/9(MGL_LOAD_TIMEOUT)
  Comms Timeout Logic/3(NG_LOAD_TIMEOUT) -> Health Check/10(NG_LOAD_TIMEOUT)
  Comms Timeout Logic/4(MGR_FLAG_TIMEOUT) -> Health Check/11(MGR_FLAG_TIMEOUT)
  Comms Timeout Logic/5(MGL_FLAG_TIMEOUT) -> Health Check/12(MGL_FLAG_TIMEOUT)
  Comms Timeout Logic/6(NG_FLAG_TIMEOUT) -> Health Check/13(NG_FLAG_TIMEOUT)
  Bus Assignment/1 -> " Output Formatting"/7(MGR_HEALTH)
  Bus Assignment1/1 -> " Output Formatting"/8(MGL_HEALTH)
  Bus Assignment2/1 -> " Output Formatting"/9(NG_HEALTH)
  Comms Timeout Logic/7(MGR_ACTIVE) -> AND/3, Bus Assignment/2
  Comms Timeout Logic/8(MGL_ACTIVE) -> AND2/3, Bus Assignment1/2
  Comms Timeout Logic/9(NG_ACTIVE) -> Bus Assignment2/2, AND3/3

== system Lib_Piccolo/Ground Detection Systems/WoW Wrapper/Variant Subsystem/Load Cell WoW Model 20/WOW Module/T//O Configuration ==
  note: Unlike when landing our persistance and latching is inverted relative to Weight Off both gears.
      |
      | Protection against WOW Failure. In the Event of a Sensor Failure and AC lift's off, NZ threshold overides WOW signal.
  WOW_Filt : Inport
  DSC_Fail : Inport  Port=2
  AND : Logic  IconShape=distinctive  AllPortsSameDT=off  OutDataTypeStr=boolean
  Bus Selector : BusSelector  OutputSignals=WOW_Filt_NG_N,WOW_Filt_MGL_N,WOW_Filt_MGR_N
  Bus Selector1 : BusSelector  OutputSignals=MGR_DSC_FAIL,MGL_DSC_FAIL
  Compare To Constant1 : simulink/Logic and Bit Operations/Compare To Constant  relop=<  const=SensorModel.WOW.Cell.TO_loadThreshold_N  OutDataTypeStr=uint8
  Compare To Constant2 : simulink/Logic and Bit Operations/Compare To Constant  relop=<  const=SensorModel.WOW.Cell.TO_loadThreshold_N  OutDataTypeStr=uint8
  Input Selection (Failure Handling) : $bdroot/Ground Detection Systems/WoW Wrapper/Variant Subsystem/Load Cell WoW Model 20/WOW Module/Landing Configuration/Input Selection (Failure Handling)  SystemSampleTime=-1
  Latch : Subsystem
  Latch Timer : Subsystem  mask{period=SensorModel.WOW.Cell.TO_latchTime_s}
      mask prompts: period "Period [s]"
  NOT : Logic  Operator=NOT  IconShape=distinctive  AllPortsSameDT=off  OutDataTypeStr=boolean
  NOT2 : Logic  Operator=NOT  IconShape=distinctive  AllPortsSameDT=off  OutDataTypeStr=boolean
  Persistance Timer : Subsystem  mask{period=SensorModel.WOW.Cell.TO_persistanceTime_s}
      mask prompts: period "Period [s]"
  Terminator : Terminator
  Unit Delay : UnitDelay  SampleTime=-1
  ContactBool : Outport
  Takeoff_Fail_L : Outport  Port=2
  Takeoff_Fail_R : Outport  Port=3
  wires:
  NOT2/1 -> ContactBool/1
  Persistance Timer/1(Expired) -> Latch/1(D)
  Compare To Constant2/1 -> AND/1
  Latch Timer/1(Expired) -> NOT/1
  Unit Delay/1 -> Latch Timer/1(Enable/!Rst)
  Compare To Constant1/1 -> AND/2
  AND/1 -> Persistance Timer/1(Enable/!Rst)
  Latch/1(Q_Latched) -> NOT2/1, Unit Delay/1  "ContactBool"
  NOT/1 -> Latch/2(Enable/!Rst)
  WOW_Filt/1 -> Bus Selector/1
  Bus Selector/1 -> Terminator/1  "<WOW_Filt_NG_N>"
  Bus Selector/2 -> Input Selection (Failure Handling)/1  "<WOW_Filt_MGL_N>"
  Bus Selector/3 -> Input Selection (Failure Handling)/2  "<WOW_Filt_MGR_N>"
  DSC_Fail/1 -> Bus Selector1/1
  Bus Selector1/1 -> Input Selection (Failure Handling)/3  "<MGR_DSC_FAIL>"
  Bus Selector1/2 -> Input Selection (Failure Handling)/4  "<MGL_DSC_FAIL>"
  Input Selection (Failure Handling)/1 -> Compare To Constant2/1  "InputL"
  Input Selection (Failure Handling)/2 -> Compare To Constant1/1  "InputR"
  Input Selection (Failure Handling)/3 -> Takeoff_Fail_L/1
  Input Selection (Failure Handling)/4 -> Takeoff_Fail_R/1

== system Lib_Piccolo/Ground Detection Systems/WoW Wrapper/Variant Subsystem/Load Cell WoW Model 20/WOW Module/Tare ==
  note: Use DSC health information to select tare value.
      |
      | If DSC is failed, use previous tare value (don't update).
      |
      | Else, sample LPF for that channel and update tare value.
  WOW_Bias_Filt_N : Inport
  DSC_Fail : Inport  Port=2
  Tare_In : Inport  Port=3
  Trigger : TriggerPort  VariantControl=Variant  PortDimensions=1
  Bus Selector : BusSelector  OutputSignals=Bias_NG_N,Bias_MGL_N,Bias_MGR_N
  Bus Selector1 : BusSelector  OutputSignals=NG_DSC_FAIL,MGL_DSC_FAIL,MGR_DSC_FAIL
  Bus Selector2 : BusSelector  OutputSignals=NG_TARE_N,MGL_TARE_N,MGR_TARE_N
  Switch : Switch  Criteria=u2 > Threshold  Threshold=0.5
  Switch1 : Switch  Criteria=u2 > Threshold  Threshold=0.5
  Switch2 : Switch  Criteria=u2 > Threshold  Threshold=0.5
  NG_TARE_N : Outport  OutDataTypeStr=single
  MGL_TARE_N : Outport  Port=2  OutDataTypeStr=single
  MGR_TARE_N : Outport  Port=3  OutDataTypeStr=single
  wires:
  WOW_Bias_Filt_N/1 -> Bus Selector/1
  Bus Selector/1 -> [Bias_NG_N]  "<Bias_NG_N>"
  Bus Selector/2 -> [Bias_MGL_N]  "<Bias_MGL_N>"
  Bus Selector/3 -> [Bias_MGR_N]  "<Bias_MGR_N>"
  DSC_Fail/1 -> Bus Selector1/1
  Bus Selector1/3 -> Switch2/2  "<MGR_DSC_FAIL>"
  Bus Selector1/2 -> Switch1/2  "<MGL_DSC_FAIL>"
  Bus Selector1/1 -> Switch/2  "<NG_DSC_FAIL>"
  Tare_In/1 -> Bus Selector2/1
  Bus Selector2/1 -> [NG_TARE]  "<NG_TARE_N>"
  Bus Selector2/2 -> [MGL_TARE]  "<MGL_TARE_N>"
  Bus Selector2/3 -> [MGR_TARE]  "<MGR_TARE_N>"
  [NG_TARE] -> Switch/1
  Switch/1 -> NG_TARE_N/1
  [Bias_NG_N] -> Switch/3
  Switch1/1 -> MGL_TARE_N/1
  [Bias_MGL_N] -> Switch1/3
  [MGL_TARE] -> Switch1/1
  [MGR_TARE] -> Switch2/1
  [Bias_MGR_N] -> Switch2/3
  Switch2/1 -> MGR_TARE_N/1

== system Lib_Piccolo/WOW Archive Container/Load Cell WoW Model 3 - LiftOff Delay/Landing Configuration/Latch Timer Selection/Latch Timer Selection/Timer Select Latch ==
  D : Inport
  Enable/!Rst : Inport  Port=2
  AND : Logic  IconShape=distinctive  AllPortsSameDT=off  OutDataTypeStr=boolean
  Constant : Constant
  OR : Logic  Operator=OR  IconShape=distinctive  AllPortsSameDT=off  OutDataTypeStr=boolean
  Switch : Switch  Criteria=u2 > Threshold  Threshold=0.5
  Unit Delay : UnitDelay  SampleTime=-1
  Q_Latched : Outport
  wires:
  Constant/1 -> Switch/1
  Enable/!Rst/1 -> AND/2
  AND/1 -> Switch/2
  OR/1 -> AND/1
  D/1 -> OR/1, Switch/3
  Switch/1 -> Unit Delay/1, Q_Latched/1
  Unit Delay/1 -> OR/2

== system Lib_Piccolo/WOW Archive Container/Load Cell WoW Model 3 - LiftOff Delay/Landing Configuration1/Latch Timer Selection/Latch Timer Selection/Timer Select Latch ==
  D : Inport
  Enable/!Rst : Inport  Port=2
  AND : Logic  IconShape=distinctive  AllPortsSameDT=off  OutDataTypeStr=boolean
  Constant : Constant
  OR : Logic  Operator=OR  IconShape=distinctive  AllPortsSameDT=off  OutDataTypeStr=boolean
  Switch : Switch  Criteria=u2 > Threshold  Threshold=0.5
  Unit Delay : UnitDelay  SampleTime=-1
  Q_Latched : Outport
  wires:
  Constant/1 -> Switch/1
  Enable/!Rst/1 -> AND/2
  AND/1 -> Switch/2
  OR/1 -> AND/1
  D/1 -> OR/1, Switch/3
  Switch/1 -> Unit Delay/1, Q_Latched/1
  Unit Delay/1 -> OR/2

== system Lib_Piccolo/WOW Archive Container/Load Cell WoW Model 4 - LiftOff Delay variation 2/Landing Configuration/Latch Timer Selection/Latch Timer Selection/Timer Select Latch ==
  D : Inport
  Enable/!Rst : Inport  Port=2
  AND : Logic  IconShape=distinctive  AllPortsSameDT=off  OutDataTypeStr=boolean
  Constant : Constant
  OR : Logic  Operator=OR  IconShape=distinctive  AllPortsSameDT=off  OutDataTypeStr=boolean
  Switch : Switch  Criteria=u2 > Threshold  Threshold=0.5
  Unit Delay : UnitDelay  SampleTime=-1
  Q_Latched : Outport
  wires:
  Constant/1 -> Switch/1
  Enable/!Rst/1 -> AND/2
  AND/1 -> Switch/2
  OR/1 -> AND/1
  D/1 -> OR/1, Switch/3
  Switch/1 -> Unit Delay/1, Q_Latched/1
  Unit Delay/1 -> OR/2

== system Lib_Piccolo/WOW Archive Container/Load Cell WoW Model 5 - Dynamic Timing/Landing Configuration/Latch Timer Selection/Latch Timer Selection/Timer Select Latch ==
  D : Inport
  Enable/!Rst : Inport  Port=2
  AND : Logic  IconShape=distinctive  AllPortsSameDT=off  OutDataTypeStr=boolean
  Constant : Constant
  OR : Logic  Operator=OR  IconShape=distinctive  AllPortsSameDT=off  OutDataTypeStr=boolean
  Switch : Switch  Criteria=u2 > Threshold  Threshold=0.5
  Unit Delay : UnitDelay  SampleTime=-1
  Q_Latched : Outport
  wires:
  Constant/1 -> Switch/1
  Enable/!Rst/1 -> AND/2
  AND/1 -> Switch/2
  OR/1 -> AND/1
  D/1 -> OR/1, Switch/3
  Switch/1 -> Unit Delay/1, Q_Latched/1
  Unit Delay/1 -> OR/2

== system Lib_Piccolo/Ground Detection Systems/WoW Wrapper/Variant Subsystem/Load Cell WoW Model 1/Landing Configuration/Latch Timer Selection/Latch Timer Selection ==
  ContactBool : Inport
  AND1 : Logic  Inputs=3  IconShape=distinctive  AllPortsSameDT=off  OutDataTypeStr=boolean
  Constant : Constant  Value=SensorModel.WOW.Cell.useDualTimer
  Invert Contact : simulink/Logic and Bit Operations/Compare To Constant  relop=<  const=0.5  OutDataTypeStr=boolean
  NOT : Logic  Operator=NOT  IconShape=distinctive  AllPortsSameDT=off  OutDataTypeStr=boolean
  Timer Select Latch : Subsystem
  Primary/!Secondary : Outport
  wires:
  [apModeEnable] -> Timer Select Latch/2(Enable/!Rst)
  Constant/1 -> AND1/2
  Timer Select Latch/1(Q_Latched) -> NOT/1  "Seconday/!Primary"
  Invert Contact/1 -> AND1/3
  [hasDetected] -> AND1/1
  AND1/1 -> Timer Select Latch/1(D)
  ContactBool/1 -> Invert Contact/1
  NOT/1 -> Primary/!Secondary/1  "Primary/!Secondary"

== system Lib_Piccolo/Ground Detection Systems/WoW Wrapper/Variant Subsystem/Load Cell WoW Model 1/Landing Configuration/Latch Timer Selection/Primary Latch Timer ==
  Enable/!Rst : Inport
  Compare To Constant1 : simulink/Logic and Bit Operations/Compare To Constant  relop=>  const=0  OutDataTypeStr=uint8
  Compare To Constant2 : simulink/Logic and Bit Operations/Compare To Constant  relop=>=  const=period  OutDataTypeStr=uint8
  Compare To Constant3 : simulink/Logic and Bit Operations/Compare To Constant  relop===  const=0  OutDataTypeStr=boolean
  Discrete-Time Integrator : DiscreteIntegrator  ExternalReset=level  SampleTime=-1  OutDataTypeStr=double  ICPrevOutput=DiscIntNeverNeededParam  ICPrevScaledInput=DiscIntNeverNeededParam
  Expired : Outport
  wires:
  Compare To Constant3/1 -> Discrete-Time Integrator/2
  Enable/!Rst/1 -> Compare To Constant3/1, Compare To Constant1/1
  Discrete-Time Integrator/1 -> Compare To Constant2/1
  Compare To Constant2/1 -> Expired/1
  Compare To Constant1/1 -> Discrete-Time Integrator/1

== system Lib_Piccolo/Ground Detection Systems/WoW Wrapper/Variant Subsystem/Load Cell WoW Model 1/Landing Configuration/Latch Timer Selection/Secondary Latch Timer ==
  Enable/!Rst : Inport
  Compare To Constant2 : simulink/Logic and Bit Operations/Compare To Constant  relop=>=  const=period  OutDataTypeStr=uint8
  Discrete-Time Integrator : DiscreteIntegrator  ExternalReset=level  SampleTime=-1  OutDataTypeStr=double  ICPrevOutput=DiscIntNeverNeededParam  ICPrevScaledInput=DiscIntNeverNeededParam
  NOT1 : Logic  Operator=NOT  IconShape=distinctive  AllPortsSameDT=off  OutDataTypeStr=boolean
  Expired : Outport
  wires:
  NOT1/1 -> Discrete-Time Integrator/2
  Discrete-Time Integrator/1 -> Compare To Constant2/1  "sTime_s"
  Compare To Constant2/1 -> Expired/1
  Enable/!Rst/1 -> Discrete-Time Integrator/1, NOT1/1

== system Lib_Piccolo/Ground Detection Systems/WoW Wrapper/Variant Subsystem/Load Cell WoW Model 1 16P5 AsFlown 2022/Landing Configuration/Latch Timer Selection/Latch Timer Selection ==
  ContactBool : Inport
  AND1 : Logic  Inputs=3  IconShape=distinctive  AllPortsSameDT=off  OutDataTypeStr=boolean
  Constant : Constant  Value=0
  Invert Contact : simulink/Logic and Bit Operations/Compare To Constant  relop=<  const=0.5  OutDataTypeStr=boolean
  NOT : Logic  Operator=NOT  IconShape=distinctive  AllPortsSameDT=off  OutDataTypeStr=boolean
  Timer Select Latch : Subsystem
  Primary/!Secondary : Outport
  wires:
  NOT/1 -> Primary/!Secondary/1  "Primary/!Secondary"
  ContactBool/1 -> Invert Contact/1
  AND1/1 -> Timer Select Latch/1(D)
  [hasDetected] -> AND1/1
  Invert Contact/1 -> AND1/3
  Timer Select Latch/1(Q_Latched) -> NOT/1  "Seconday/!Primary"
  Constant/1 -> AND1/2
  [apModeEnable] -> Timer Select Latch/2(Enable/!Rst)

== system Lib_Piccolo/Ground Detection Systems/WoW Wrapper/Variant Subsystem/Load Cell WoW Model 1 16P5 AsFlown 2022/Landing Configuration/Latch Timer Selection/Primary Latch Timer ==
  Enable/!Rst : Inport
  Compare To Constant1 : simulink/Logic and Bit Operations/Compare To Constant  relop=>  const=0  OutDataTypeStr=uint8
  Compare To Constant2 : simulink/Logic and Bit Operations/Compare To Constant  relop=>=  const=period  OutDataTypeStr=uint8
  Compare To Constant3 : simulink/Logic and Bit Operations/Compare To Constant  relop===  const=0  OutDataTypeStr=boolean
  Discrete-Time Integrator : DiscreteIntegrator  ExternalReset=level  SampleTime=-1  OutDataTypeStr=double  ICPrevOutput=DiscIntNeverNeededParam  ICPrevScaledInput=DiscIntNeverNeededParam
  Expired : Outport
  wires:
  Compare To Constant1/1 -> Discrete-Time Integrator/1
  Compare To Constant2/1 -> Expired/1
  Discrete-Time Integrator/1 -> Compare To Constant2/1
  Enable/!Rst/1 -> Compare To Constant1/1, Compare To Constant3/1
  Compare To Constant3/1 -> Discrete-Time Integrator/2

== system Lib_Piccolo/Ground Detection Systems/WoW Wrapper/Variant Subsystem/Load Cell WoW Model 1 16P5 AsFlown 2022/Landing Configuration/Latch Timer Selection/Secondary Latch Timer ==
  Enable/!Rst : Inport
  Compare To Constant2 : simulink/Logic and Bit Operations/Compare To Constant  relop=>=  const=period  OutDataTypeStr=uint8
  Discrete-Time Integrator : DiscreteIntegrator  ExternalReset=level  SampleTime=-1  OutDataTypeStr=double  ICPrevOutput=DiscIntNeverNeededParam  ICPrevScaledInput=DiscIntNeverNeededParam
  NOT1 : Logic  Operator=NOT  IconShape=distinctive  AllPortsSameDT=off  OutDataTypeStr=boolean
  Expired : Outport
  wires:
  Enable/!Rst/1 -> NOT1/1, Discrete-Time Integrator/1
  Compare To Constant2/1 -> Expired/1
  Discrete-Time Integrator/1 -> Compare To Constant2/1  "sTime_s"
  NOT1/1 -> Discrete-Time Integrator/2

== system Lib_Piccolo/Ground Detection Systems/WoW Wrapper/Variant Subsystem/Load Cell WoW Model 1 7P AsFlown/Landing Configuration/Latch Timer Selection/Latch Timer Selection ==
  ContactBool : Inport
  AND1 : Logic  Inputs=3  IconShape=distinctive  AllPortsSameDT=off  OutDataTypeStr=boolean
  Constant : Constant  Value=0
  Invert Contact : simulink/Logic and Bit Operations/Compare To Constant  relop=<  const=0.5  OutDataTypeStr=boolean
  NOT : Logic  Operator=NOT  IconShape=distinctive  AllPortsSameDT=off  OutDataTypeStr=boolean
  Timer Select Latch : Subsystem
  Primary/!Secondary : Outport
  wires:
  [apModeEnable] -> Timer Select Latch/2(Enable/!Rst)
  Constant/1 -> AND1/2
  Timer Select Latch/1(Q_Latched) -> NOT/1  "Seconday/!Primary"
  Invert Contact/1 -> AND1/3
  [hasDetected] -> AND1/1
  AND1/1 -> Timer Select Latch/1(D)
  ContactBool/1 -> Invert Contact/1
  NOT/1 -> Primary/!Secondary/1  "Primary/!Secondary"
